simulink model "CombinedExperiment"  (R2020a)
settings: Solver=FixedStepAuto  StartTime=0.0  StopTime=tsim  FixedStep=baseRate  RelTol=1e-3  EnableMultiTasking=on
values from neighbouring files (symbols this model uses):
  baseRate = 0.1    [Run_Initializer.m]
  drop_states_BLACK = [1.36947387695313,1.22175756835938,-0.0161599479615688]    [Run_Initializer.m]
  drop_states_BLUE = [ xLength/2+0.9; yLength/2+0.5; 0]    [Run_Initializer.m]
  drop_states_RED = [ xLength/2+1.1; yLength/2; pi]    [Run_Initializer.m]
  F_thrusters_BLACK = 0.25.*ones(8,1)    [Run_Initializer.m]
  F_thrusters_BLUE = 0.25.*ones(8,1)    [Run_Initializer.m]
  F_thrusters_RED = 0.25.*ones(8,1)    [Run_Initializer.m]
  home_states_BLACK = [ xLength/2; yLength/2; 0]    [Run_Initializer.m]
  home_states_BLUE = [ xLength/2-0.9; yLength/2+0.5; 0]    [Run_Initializer.m]
  home_states_RED = [ xLength/2+1.1; yLength/2; pi]    [Run_Initializer.m]
  init_states_BLACK = [ xLength/2; yLength/2; 0]    [Run_Initializer.m]
  init_states_BLUE = [ xLength/2+0.9; yLength/2+0.5; 0]    [Run_Initializer.m]
  init_states_RED = [ xLength/2+1.1; yLength/2; pi]    [Run_Initializer.m]
  Kd_tb = 0.4    [Run_Initializer.m]
  Kd_tblue = 0.4    [Run_Initializer.m]
  Kd_tr = 0.4    [Run_Initializer.m]
  Kd_xb = 5    [Run_Initializer.m]
  Kd_xblue = 5    [Run_Initializer.m]
  Kd_xr = 5    [Run_Initializer.m]
  Kd_yb = 5    [Run_Initializer.m]
  Kd_yblue = 5    [Run_Initializer.m]
  Kd_yr = 5    [Run_Initializer.m]
  Kp_tb = 0.1    [Run_Initializer.m]
  Kp_tblue = 0.1    [Run_Initializer.m]
  Kp_tr = 0.1    [Run_Initializer.m]
  Kp_xb = 2    [Run_Initializer.m]
  Kp_xblue = 2    [Run_Initializer.m]
  Kp_xr = 2    [Run_Initializer.m]
  Kp_yb = 2    [Run_Initializer.m]
  Kp_yblue = 2    [Run_Initializer.m]
  Kp_yr = 2    [Run_Initializer.m]
  noise_variance_BLACK = 0    [Run_Initializer.m]
  noise_variance_BLUE = 0    [Run_Initializer.m]
  noise_variance_RED = 0    [Run_Initializer.m]
  Phase0_End = Phase0_Duration    (= 10)    [Run_Initializer.m]
  Phase1_End = Phase0_Duration + Phase1_Duration    (= 15)    [Run_Initializer.m]
  Phase2_End = Phase0_Duration + Phase1_Duration +                                   Phase2_Duration    (= 40)    [Run_Initializer.m]
  Phase3_End = Phase0_Duration + Phase1_Duration +                                   Phase2_Duration + Phase3_Duration    (= 117)    [Run_Initializer.m]
  Phase3_SubPhase1_End = Phase2_End + Phase3_SubPhase1_Duration    (= 41)    [Run_Initializer.m]
  Phase3_SubPhase2_End = Phase2_End + Phase3_SubPhase1_Duration +                                   Phase3_SubPhase2_Duration    (= 42)    [Run_Initializer.m]
  Phase3_SubPhase3_End = Phase2_End + Phase3_SubPhase1_Duration +                                   Phase3_SubPhase2_Duration +                                  Phase3_SubPhase3_Duration    (= 72)    [Run_Initializer.m]
  Phase3_SubPhase4_End = Phase2_End + Phase3_SubPhase1_Duration +                                   Phase3_SubPhase2_Duration +                                  Phase3_SubPhase3_Duration +                                  Phase3_SubPhase4_Duration    [Run_Initializer.m]
  Phase4_End = Phase0_Duration + Phase1_Duration +                                   Phase2_Duration + Phase3_Duration +                                   Phase4_Duration    (= 137)    [Run_Initializer.m]
  Phase5_End = Phase0_Duration + Phase1_Duration +                                   Phase2_Duration + Phase3_Duration +                                   Phase4_Duration + Phase5_Duration    (= 142)    [Run_Initializer.m]
  serverRate = 0.2    [Run_Initializer.m]
  thruster_dist2CG_BLACK = [83.42;-52.58;55.94;-60.05;54.08;-53.92;77.06;-55.94]    [Run_Initializer.m]
  thruster_dist2CG_BLUE = [83.42;-52.58;55.94;-60.05;54.08;-53.92;77.06;-55.94]    [Run_Initializer.m]
  thruster_dist2CG_RED = [49.92;-78.08;70.46;-63.54;81.08;-50.42;57.44;-75.96]    [Run_Initializer.m]
  xLength = 3.51155    [Run_Initializer.m]
  yLength = 2.41935    [Run_Initializer.m]
undefined symbols (not defined in the file or in its folder): DiscIntNeverNeededParam, platformSelection, simMode, WhoAmI
libraries: dspstat3 x18, raspberrypiBasiclib x10, dspsigops x9, embdlinuxlib x8, simulink x8, MainLibrary x5, mspfiltlib x3, dsparch4 x3, dspswit3 x2, sensehatlib x1
(part 8 of 9)

== system CombinedExperiment/Gyroscope & Acceleration Algorithms/Change BLUE Behavior/Fix Initial Bias (Accel)/Correct AccelZ/Subsystem ==
  Universal_Time : DataStoreRead  DataStoreName=Univ_Time
  Time : Outport  VectorParamsAs1DForOutWhenUnconnected=off
  wires:
  Universal_Time/1 -> Time/1

== system CombinedExperiment/Gyroscope & Acceleration Algorithms/Change RED Behavior/Fix Initial Bias/Correct GyroX/Calculate Running Mean ==
  In1 : Inport
  Action Port : ActionPort  ActionPortLabel=if(u1 < 5)
  Delay : Delay  DelayLength=1
  Delay1 : Delay
  Delay2 : Delay  DelayLength=4
  Delay3 : Delay  DelayLength=5
  Delay4 : Delay  DelayLength=3
  Mean : dspstat3/Mean  run=off  InputProcessing=Columns as channels (frame based)  reset_popup=None  directionMode=Each column  dimension=1  roiEnable=off  roiType=Rectangles  roiPortion=Entire ROI  roiOutput=Individual statistics for each ROI  roiFlag=off  roundingMode=Floor  overflowMode=off  outputDataTypeStr=Inherit: Same as accumulator  outputMin=[]  outputMax=[]  outputLastDataTypeStr=Inherit: Same as accumulator
  Mux : Mux  Inputs=6
  Out1 : Outport
  wires:
  Delay3/1 -> Mux/6
  Delay2/1 -> Mux/5
  Delay1/1 -> Mux/3
  Delay4/1 -> Mux/4
  Delay/1 -> Mux/2
  In1/1 -> Delay3/1, Delay2/1, Delay4/1, Delay1/1, Delay/1, Mux/1
  Mux/1 -> Mean/1
  Mean/1 -> Out1/1

== system CombinedExperiment/Gyroscope & Acceleration Algorithms/Change RED Behavior/Fix Initial Bias/Correct GyroX/Pass Current Gyro ==
  In1 : Inport
  Action Port : ActionPort  ActionPortLabel=else
  Out1 : Outport
  wires:
  In1/1 -> Out1/1

== system CombinedExperiment/Gyroscope & Acceleration Algorithms/Change RED Behavior/Fix Initial Bias/Correct GyroX/Subsystem ==
  Universal_Time : DataStoreRead  DataStoreName=Univ_Time
  Time : Outport  VectorParamsAs1DForOutWhenUnconnected=off
  wires:
  Universal_Time/1 -> Time/1

== system CombinedExperiment/Gyroscope & Acceleration Algorithms/Change RED Behavior/Fix Initial Bias/Correct GyroY/Calculate Running Mean ==
  In1 : Inport
  Action Port : ActionPort  ActionPortLabel=if(u1 < 5)
  Delay : Delay  DelayLength=1
  Delay1 : Delay
  Delay2 : Delay  DelayLength=4
  Delay3 : Delay  DelayLength=5
  Delay4 : Delay  DelayLength=3
  Mean : dspstat3/Mean  run=off  InputProcessing=Columns as channels (frame based)  reset_popup=None  directionMode=Each column  dimension=1  roiEnable=off  roiType=Rectangles  roiPortion=Entire ROI  roiOutput=Individual statistics for each ROI  roiFlag=off  roundingMode=Floor  overflowMode=off  outputDataTypeStr=Inherit: Same as accumulator  outputMin=[]  outputMax=[]  outputLastDataTypeStr=Inherit: Same as accumulator
  Mux : Mux  Inputs=6
  Out1 : Outport
  wires:
  Delay3/1 -> Mux/6
  Delay2/1 -> Mux/5
  Delay1/1 -> Mux/3
  Delay4/1 -> Mux/4
  Delay/1 -> Mux/2
  In1/1 -> Delay3/1, Delay2/1, Delay4/1, Delay1/1, Delay/1, Mux/1
  Mux/1 -> Mean/1
  Mean/1 -> Out1/1

== system CombinedExperiment/Gyroscope & Acceleration Algorithms/Change RED Behavior/Fix Initial Bias/Correct GyroY/Pass Current Gyro ==
  In1 : Inport
  Action Port : ActionPort  ActionPortLabel=else
  Out1 : Outport
  wires:
  In1/1 -> Out1/1

== system CombinedExperiment/Gyroscope & Acceleration Algorithms/Change RED Behavior/Fix Initial Bias/Correct GyroY/Subsystem ==
  Universal_Time : DataStoreRead  DataStoreName=Univ_Time
  Time : Outport  VectorParamsAs1DForOutWhenUnconnected=off
  wires:
  Universal_Time/1 -> Time/1

== system CombinedExperiment/Gyroscope & Acceleration Algorithms/Change RED Behavior/Fix Initial Bias/Correct GyroZ/Calculate Running Mean ==
  In1 : Inport
  Action Port : ActionPort  ActionPortLabel=if(u1 < 5)
  Delay : Delay  DelayLength=1
  Delay1 : Delay
  Delay2 : Delay  DelayLength=4
  Delay3 : Delay  DelayLength=5
  Delay4 : Delay  DelayLength=3
  Mean : dspstat3/Mean  run=off  InputProcessing=Columns as channels (frame based)  reset_popup=None  directionMode=Each column  dimension=1  roiEnable=off  roiType=Rectangles  roiPortion=Entire ROI  roiOutput=Individual statistics for each ROI  roiFlag=off  roundingMode=Floor  overflowMode=off  outputDataTypeStr=Inherit: Same as accumulator  outputMin=[]  outputMax=[]  outputLastDataTypeStr=Inherit: Same as accumulator
  Mux : Mux  Inputs=6
  Out1 : Outport
  wires:
  Delay3/1 -> Mux/6
  Delay2/1 -> Mux/5
  Delay1/1 -> Mux/3
  Delay4/1 -> Mux/4
  Delay/1 -> Mux/2
  In1/1 -> Delay3/1, Delay2/1, Delay4/1, Delay1/1, Delay/1, Mux/1
  Mux/1 -> Mean/1
  Mean/1 -> Out1/1

== system CombinedExperiment/Gyroscope & Acceleration Algorithms/Change RED Behavior/Fix Initial Bias/Correct GyroZ/Pass Current Gyro ==
  In1 : Inport
  Action Port : ActionPort  ActionPortLabel=else
  Out1 : Outport
  wires:
  In1/1 -> Out1/1

== system CombinedExperiment/Gyroscope & Acceleration Algorithms/Change RED Behavior/Fix Initial Bias/Correct GyroZ/Subsystem ==
  Universal_Time : DataStoreRead  DataStoreName=Univ_Time
  Time : Outport  VectorParamsAs1DForOutWhenUnconnected=off
  wires:
  Universal_Time/1 -> Time/1

== system CombinedExperiment/Gyroscope & Acceleration Algorithms/Change RED Behavior/Fix Initial Bias (Accel)/Correct AccelX/Calculate Running Mean ==
  In1 : Inport
  Action Port : ActionPort  ActionPortLabel=if(u1 < 5)
  Delay : Delay  DelayLength=1
  Delay1 : Delay
  Delay2 : Delay  DelayLength=4
  Delay3 : Delay  DelayLength=5
  Delay4 : Delay  DelayLength=3
  Mean : dspstat3/Mean  run=off  InputProcessing=Columns as channels (frame based)  reset_popup=None  directionMode=Each column  dimension=1  roiEnable=off  roiType=Rectangles  roiPortion=Entire ROI  roiOutput=Individual statistics for each ROI  roiFlag=off  roundingMode=Floor  overflowMode=off  outputDataTypeStr=Inherit: Same as accumulator  outputMin=[]  outputMax=[]  outputLastDataTypeStr=Inherit: Same as accumulator
  Mux : Mux  Inputs=6
  Out1 : Outport
  wires:
  Delay3/1 -> Mux/6
  Delay2/1 -> Mux/5
  Delay1/1 -> Mux/3
  Delay4/1 -> Mux/4
  Delay/1 -> Mux/2
  In1/1 -> Delay3/1, Delay2/1, Delay4/1, Delay1/1, Delay/1, Mux/1
  Mux/1 -> Mean/1
  Mean/1 -> Out1/1

== system CombinedExperiment/Gyroscope & Acceleration Algorithms/Change RED Behavior/Fix Initial Bias (Accel)/Correct AccelX/Pass Current Accel ==
  In1 : Inport
  Action Port : ActionPort  ActionPortLabel=else
  Out1 : Outport
  wires:
  In1/1 -> Out1/1

== system CombinedExperiment/Gyroscope & Acceleration Algorithms/Change RED Behavior/Fix Initial Bias (Accel)/Correct AccelX/Subsystem ==
  Universal_Time : DataStoreRead  DataStoreName=Univ_Time
  Time : Outport  VectorParamsAs1DForOutWhenUnconnected=off
  wires:
  Universal_Time/1 -> Time/1

== system CombinedExperiment/Gyroscope & Acceleration Algorithms/Change RED Behavior/Fix Initial Bias (Accel)/Correct AccelY/Calculate Running Mean ==
  In1 : Inport
  Action Port : ActionPort  ActionPortLabel=if(u1 < 5)
  Delay : Delay  DelayLength=1
  Delay1 : Delay
  Delay2 : Delay  DelayLength=4
  Delay3 : Delay  DelayLength=5
  Delay4 : Delay  DelayLength=3
  Mean : dspstat3/Mean  run=off  InputProcessing=Columns as channels (frame based)  reset_popup=None  directionMode=Each column  dimension=1  roiEnable=off  roiType=Rectangles  roiPortion=Entire ROI  roiOutput=Individual statistics for each ROI  roiFlag=off  roundingMode=Floor  overflowMode=off  outputDataTypeStr=Inherit: Same as accumulator  outputMin=[]  outputMax=[]  outputLastDataTypeStr=Inherit: Same as accumulator
  Mux : Mux  Inputs=6
  Out1 : Outport
  wires:
  Delay3/1 -> Mux/6
  Delay2/1 -> Mux/5
  Delay1/1 -> Mux/3
  Delay4/1 -> Mux/4
  Delay/1 -> Mux/2
  In1/1 -> Delay3/1, Delay2/1, Delay4/1, Delay1/1, Delay/1, Mux/1
  Mux/1 -> Mean/1
  Mean/1 -> Out1/1

== system CombinedExperiment/Gyroscope & Acceleration Algorithms/Change RED Behavior/Fix Initial Bias (Accel)/Correct AccelY/Pass Current Accel ==
  In1 : Inport
  Action Port : ActionPort  ActionPortLabel=else
  Out1 : Outport
  wires:
  In1/1 -> Out1/1

== system CombinedExperiment/Gyroscope & Acceleration Algorithms/Change RED Behavior/Fix Initial Bias (Accel)/Correct AccelY/Subsystem ==
  Universal_Time : DataStoreRead  DataStoreName=Univ_Time
  Time : Outport  VectorParamsAs1DForOutWhenUnconnected=off
  wires:
  Universal_Time/1 -> Time/1

== system CombinedExperiment/Gyroscope & Acceleration Algorithms/Change RED Behavior/Fix Initial Bias (Accel)/Correct AccelZ/Calculate Running Mean ==
  In1 : Inport
  Action Port : ActionPort  ActionPortLabel=if(u1 < 5)
  Constant : Constant  Value=9.81
  Delay : Delay  DelayLength=1
  Delay1 : Delay
  Delay2 : Delay  DelayLength=4
  Delay3 : Delay  DelayLength=5
  Delay4 : Delay  DelayLength=3
  Mean : dspstat3/Mean  run=off  InputProcessing=Columns as channels (frame based)  reset_popup=None  directionMode=Each column  dimension=1  roiEnable=off  roiType=Rectangles  roiPortion=Entire ROI  roiOutput=Individual statistics for each ROI  roiFlag=off  roundingMode=Floor  overflowMode=off  outputDataTypeStr=Inherit: Same as accumulator  outputMin=[]  outputMax=[]  outputLastDataTypeStr=Inherit: Same as accumulator
  Mux : Mux  Inputs=6
  Subtract : Sum  Inputs=+-
  Out1 : Outport
  wires:
  Delay3/1 -> Mux/6
  Delay2/1 -> Mux/5
  Delay1/1 -> Mux/3
  Delay4/1 -> Mux/4
  Delay/1 -> Mux/2
  In1/1 -> Delay3/1, Delay2/1, Delay4/1, Delay1/1, Delay/1, Mux/1
  Mux/1 -> Mean/1
  Subtract/1 -> Out1/1
  Mean/1 -> Subtract/1
  Constant/1 -> Subtract/2

== system CombinedExperiment/Gyroscope & Acceleration Algorithms/Change RED Behavior/Fix Initial Bias (Accel)/Correct AccelZ/Pass Current Accel ==
  In1 : Inport
  Action Port : ActionPort  ActionPortLabel=else
  Out1 : Outport
  wires:
  In1/1 -> Out1/1

== system CombinedExperiment/Gyroscope & Acceleration Algorithms/Change RED Behavior/Fix Initial Bias (Accel)/Correct AccelZ/Subsystem ==
  Universal_Time : DataStoreRead  DataStoreName=Univ_Time
  Time : Outport  VectorParamsAs1DForOutWhenUnconnected=off
  wires:
  Universal_Time/1 -> Time/1

== system CombinedExperiment/Phase #2: Move to Initial Position/Change BLACK Behavior/Custom Discrete PD (Attitude)/x_dot -> x1/Hold this value ==
  In1 : Inport
  Action Port : ActionPort  ActionPortLabel=if(u1 ~= 0)
  Out1 : Outport  VectorParamsAs1DForOutWhenUnconnected=off
  wires:
  In1/1 -> Out1/1

== system CombinedExperiment/Phase #2: Move to Initial Position/Change BLACK Behavior/Custom Discrete PD (X-Position)/x_dot -> x1/Hold this value ==
  In1 : Inport
  Action Port : ActionPort  ActionPortLabel=if(u1 ~= 0)
  Out1 : Outport  VectorParamsAs1DForOutWhenUnconnected=off
  wires:
  In1/1 -> Out1/1

== system CombinedExperiment/Phase #2: Move to Initial Position/Change BLACK Behavior/Custom Discrete PD (Y-Position)/x_dot -> x1/Hold this value ==
  In1 : Inport
  Action Port : ActionPort  ActionPortLabel=if(u1 ~= 0)
  Out1 : Outport  VectorParamsAs1DForOutWhenUnconnected=off
  wires:
  In1/1 -> Out1/1

== system CombinedExperiment/Phase #2: Move to Initial Position/Change BLUE Behavior/Custom Discrete PD (Attitude)/x_dot -> x1/Hold this value ==
  In1 : Inport
  Action Port : ActionPort  ActionPortLabel=if(u1 ~= 0)
  Out1 : Outport  VectorParamsAs1DForOutWhenUnconnected=off
  wires:
  In1/1 -> Out1/1

== system CombinedExperiment/Phase #2: Move to Initial Position/Change BLUE Behavior/Custom Discrete PD (X-Position)/x_dot -> x1/Hold this value ==
  In1 : Inport
  Action Port : ActionPort  ActionPortLabel=if(u1 ~= 0)
  Out1 : Outport  VectorParamsAs1DForOutWhenUnconnected=off
  wires:
  In1/1 -> Out1/1

== system CombinedExperiment/Phase #2: Move to Initial Position/Change BLUE Behavior/Custom Discrete PD (Y-Position)/x_dot -> x1/Hold this value ==
  In1 : Inport
  Action Port : ActionPort  ActionPortLabel=if(u1 ~= 0)
  Out1 : Outport  VectorParamsAs1DForOutWhenUnconnected=off
  wires:
  In1/1 -> Out1/1

== system CombinedExperiment/Phase #2: Move to Initial Position/Change RED Behavior/Custom Discrete PD (Attitude)/x_dot -> x1/Hold this value ==
  In1 : Inport
  Action Port : ActionPort  ActionPortLabel=if(u1 ~= 0)
  Out1 : Outport  VectorParamsAs1DForOutWhenUnconnected=off
  wires:
  In1/1 -> Out1/1

== system CombinedExperiment/Phase #2: Move to Initial Position/Change RED Behavior/Custom Discrete PD (X-Position)/x_dot -> x1/Hold this value ==
  In1 : Inport
  Action Port : ActionPort  ActionPortLabel=if(u1 ~= 0)
  Out1 : Outport  VectorParamsAs1DForOutWhenUnconnected=off
  wires:
  In1/1 -> Out1/1

== system CombinedExperiment/Phase #2: Move to Initial Position/Change RED Behavior/Custom Discrete PD (Y-Position)/x_dot -> x1/Hold this value ==
  In1 : Inport
  Action Port : ActionPort  ActionPortLabel=if(u1 ~= 0)
  Out1 : Outport  VectorParamsAs1DForOutWhenUnconnected=off
  wires:
  In1/1 -> Out1/1

== system CombinedExperiment/Phase #3: Experiment/Change BLACK Behavior/Sub-Phase #1/Custom Discrete PD (Attitude)/x_dot -> x1 ==
  note: dy/dt ~= (y2-y1)/deltaT
  y(t) : Inport
  Delay1 : Delay  DelayLength=1  InitialConditionSource=Input port
      settings: InputPortMap=u0,p4
  Hold this value : Subsystem  TreatAsAtomicUnit=on
  Sum6 : Sum  Inputs=-+|
  divide by delta T : Gain  Gain=1/serverRate
  "if we went through a \"step\"" : If  IfExpression=u1 ~= 0  ShowElse=off
  dy(t)/dt : Outport  VectorParamsAs1DForOutWhenUnconnected=off
  wires:
  divide by delta T/1 -> dy(t)/dt/1
  Delay1/1 -> Sum6/1
  "if we went through a \"step\""/1 -> Hold this value/Action
  Hold this value/1(Out1) -> divide by delta T/1
  Sum6/1 -> "if we went through a \"step\""/1, Hold this value/1(In1)
  y(t)/1 -> Sum6/2, Delay1/2, Delay1/1

== system CombinedExperiment/Phase #3: Experiment/Change BLACK Behavior/Sub-Phase #1/Custom Discrete PD (X-Position)/x_dot -> x1 ==
  note: dy/dt ~= (y2-y1)/deltaT
  y(t) : Inport
  Delay1 : Delay  DelayLength=1  InitialConditionSource=Input port
      settings: InputPortMap=u0,p4
  Hold this value : Subsystem  TreatAsAtomicUnit=on
  Sum6 : Sum  Inputs=-+|
  divide by delta T : Gain  Gain=1/serverRate
  "if we went through a \"step\"" : If  IfExpression=u1 ~= 0  ShowElse=off
  dy(t)/dt : Outport  VectorParamsAs1DForOutWhenUnconnected=off
  wires:
  divide by delta T/1 -> dy(t)/dt/1
  Delay1/1 -> Sum6/1
  "if we went through a \"step\""/1 -> Hold this value/Action
  Hold this value/1(Out1) -> divide by delta T/1
  Sum6/1 -> "if we went through a \"step\""/1, Hold this value/1(In1)
  y(t)/1 -> Sum6/2, Delay1/2, Delay1/1

== system CombinedExperiment/Phase #3: Experiment/Change BLACK Behavior/Sub-Phase #1/Custom Discrete PD (Y-Position)/x_dot -> x1 ==
  note: dy/dt ~= (y2-y1)/deltaT
  y(t) : Inport
  Delay1 : Delay  DelayLength=1  InitialConditionSource=Input port
      settings: InputPortMap=u0,p4
  Hold this value : Subsystem  TreatAsAtomicUnit=on
  Sum6 : Sum  Inputs=-+|
  divide by delta T : Gain  Gain=1/serverRate
  "if we went through a \"step\"" : If  IfExpression=u1 ~= 0  ShowElse=off
  dy(t)/dt : Outport  VectorParamsAs1DForOutWhenUnconnected=off
  wires:
  divide by delta T/1 -> dy(t)/dt/1
  Delay1/1 -> Sum6/1
  "if we went through a \"step\""/1 -> Hold this value/Action
  Hold this value/1(Out1) -> divide by delta T/1
  Sum6/1 -> "if we went through a \"step\""/1, Hold this value/1(In1)
  y(t)/1 -> Sum6/2, Delay1/2, Delay1/1

== system CombinedExperiment/Phase #3: Experiment/Change BLACK Behavior/Sub-Phase #4/BLACK_RzD/Subsystem ==
  Constant1 : Constant  Value=Phase3_SubPhase3_End  SampleTime=-1
  Subtract : Sum  Inputs=+-
  Universal_Time : DataStoreRead  DataStoreName=Univ_Time
  Time : Outport  VectorParamsAs1DForOutWhenUnconnected=off
  wires:
  Universal_Time/1 -> Subtract/1
  Subtract/1 -> Time/1
  Constant1/1 -> Subtract/2

== system CombinedExperiment/Phase #3: Experiment/Change BLACK Behavior/Sub-Phase #4/BLACK_RzD/Wrap1 ==
  unwrapped : Inport
  MATLAB Function : MATLAB Function  TreatAsAtomicUnit=on
  wrapped : Outport  VectorParamsAs1DForOutWhenUnconnected=off
  wires:
  MATLAB Function/1(wrappedAngle) -> wrapped/1
  unwrapped/1 -> MATLAB Function/1(u)

== system CombinedExperiment/Phase #3: Experiment/Change BLACK Behavior/Sub-Phase #4/BLACK_RzD1/Subsystem ==
  Constant1 : Constant  Value=Phase3_SubPhase3_End  SampleTime=-1
  Subtract : Sum  Inputs=+-
  Universal_Time : DataStoreRead  DataStoreName=Univ_Time
  Time : Outport  VectorParamsAs1DForOutWhenUnconnected=off
  wires:
  Universal_Time/1 -> Subtract/1
  Subtract/1 -> Time/1
  Constant1/1 -> Subtract/2

== system CombinedExperiment/Phase #3: Experiment/Change BLACK Behavior/Sub-Phase #4/BLACK_RzD1/Wrap1 ==
  unwrapped : Inport
  MATLAB Function : MATLAB Function  TreatAsAtomicUnit=on
  wrapped : Outport  VectorParamsAs1DForOutWhenUnconnected=off
  wires:
  MATLAB Function/1(wrappedAngle) -> wrapped/1
  unwrapped/1 -> MATLAB Function/1(u)

== system CombinedExperiment/Phase #3: Experiment/Change BLACK Behavior/Sub-Phase #4/Custom Discrete PD (Attitude)/x_dot -> x1 ==
  note: dy/dt ~= (y2-y1)/deltaT
  y(t) : Inport
  Delay1 : Delay  DelayLength=1  InitialConditionSource=Input port
      settings: InputPortMap=u0,p4
  Hold this value : Subsystem  TreatAsAtomicUnit=on
  Sum6 : Sum  Inputs=-+|
  divide by delta T : Gain  Gain=1/serverRate
  "if we went through a \"step\"" : If  IfExpression=u1 ~= 0  ShowElse=off
  dy(t)/dt : Outport  VectorParamsAs1DForOutWhenUnconnected=off
  wires:
  divide by delta T/1 -> dy(t)/dt/1
  Delay1/1 -> Sum6/1
  "if we went through a \"step\""/1 -> Hold this value/Action
  Hold this value/1(Out1) -> divide by delta T/1
  Sum6/1 -> "if we went through a \"step\""/1, Hold this value/1(In1)
  y(t)/1 -> Sum6/2, Delay1/2, Delay1/1

== system CombinedExperiment/Phase #3: Experiment/Change BLACK Behavior/Sub-Phase #4/Custom Discrete PD (X-Position)/x_dot -> x1 ==
  note: dy/dt ~= (y2-y1)/deltaT
  y(t) : Inport
  Delay1 : Delay  DelayLength=1  InitialConditionSource=Input port
      settings: InputPortMap=u0,p4
  Hold this value : Subsystem  TreatAsAtomicUnit=on
  Sum6 : Sum  Inputs=-+|
  divide by delta T : Gain  Gain=1/serverRate
  "if we went through a \"step\"" : If  IfExpression=u1 ~= 0  ShowElse=off
  dy(t)/dt : Outport  VectorParamsAs1DForOutWhenUnconnected=off
  wires:
  divide by delta T/1 -> dy(t)/dt/1
  Delay1/1 -> Sum6/1
  "if we went through a \"step\""/1 -> Hold this value/Action
  Hold this value/1(Out1) -> divide by delta T/1
  Sum6/1 -> "if we went through a \"step\""/1, Hold this value/1(In1)
  y(t)/1 -> Sum6/2, Delay1/2, Delay1/1

== system CombinedExperiment/Phase #3: Experiment/Change BLACK Behavior/Sub-Phase #4/Custom Discrete PD (Y-Position)/x_dot -> x1 ==
  note: dy/dt ~= (y2-y1)/deltaT
  y(t) : Inport
  Delay1 : Delay  DelayLength=1  InitialConditionSource=Input port
      settings: InputPortMap=u0,p4
  Hold this value : Subsystem  TreatAsAtomicUnit=on
  Sum6 : Sum  Inputs=-+|
  divide by delta T : Gain  Gain=1/serverRate
  "if we went through a \"step\"" : If  IfExpression=u1 ~= 0  ShowElse=off
  dy(t)/dt : Outport  VectorParamsAs1DForOutWhenUnconnected=off
  wires:
  divide by delta T/1 -> dy(t)/dt/1
  Delay1/1 -> Sum6/1
  "if we went through a \"step\""/1 -> Hold this value/Action
  Hold this value/1(Out1) -> divide by delta T/1
  Sum6/1 -> "if we went through a \"step\""/1, Hold this value/1(In1)
  y(t)/1 -> Sum6/2, Delay1/2, Delay1/1

== system CombinedExperiment/Phase #3: Experiment/Change BLUE Behavior/Sub-Phase #1/Custom Discrete PD (Attitude)/x_dot -> x1 ==
  note: dy/dt ~= (y2-y1)/deltaT
  y(t) : Inport
  Delay1 : Delay  DelayLength=1  InitialConditionSource=Input port
      settings: InputPortMap=u0,p4
  Hold this value : Subsystem  TreatAsAtomicUnit=on
  Sum6 : Sum  Inputs=-+|
  divide by delta T : Gain  Gain=1/serverRate
  "if we went through a \"step\"" : If  IfExpression=u1 ~= 0  ShowElse=off
  dy(t)/dt : Outport  VectorParamsAs1DForOutWhenUnconnected=off
  wires:
  divide by delta T/1 -> dy(t)/dt/1
  Delay1/1 -> Sum6/1
  "if we went through a \"step\""/1 -> Hold this value/Action
  Hold this value/1(Out1) -> divide by delta T/1
  Sum6/1 -> "if we went through a \"step\""/1, Hold this value/1(In1)
  y(t)/1 -> Sum6/2, Delay1/2, Delay1/1

== system CombinedExperiment/Phase #3: Experiment/Change BLUE Behavior/Sub-Phase #1/Custom Discrete PD (X-Position)/x_dot -> x1 ==
  note: dy/dt ~= (y2-y1)/deltaT
  y(t) : Inport
  Delay1 : Delay  DelayLength=1  InitialConditionSource=Input port
      settings: InputPortMap=u0,p4
  Hold this value : Subsystem  TreatAsAtomicUnit=on
  Sum6 : Sum  Inputs=-+|
  divide by delta T : Gain  Gain=1/serverRate
  "if we went through a \"step\"" : If  IfExpression=u1 ~= 0  ShowElse=off
  dy(t)/dt : Outport  VectorParamsAs1DForOutWhenUnconnected=off
  wires:
  divide by delta T/1 -> dy(t)/dt/1
  Delay1/1 -> Sum6/1
  "if we went through a \"step\""/1 -> Hold this value/Action
  Hold this value/1(Out1) -> divide by delta T/1
  Sum6/1 -> "if we went through a \"step\""/1, Hold this value/1(In1)
  y(t)/1 -> Sum6/2, Delay1/2, Delay1/1

== system CombinedExperiment/Phase #3: Experiment/Change BLUE Behavior/Sub-Phase #1/Custom Discrete PD (Y-Position)/x_dot -> x1 ==
  note: dy/dt ~= (y2-y1)/deltaT
  y(t) : Inport
  Delay1 : Delay  DelayLength=1  InitialConditionSource=Input port
      settings: InputPortMap=u0,p4
  Hold this value : Subsystem  TreatAsAtomicUnit=on
  Sum6 : Sum  Inputs=-+|
  divide by delta T : Gain  Gain=1/serverRate
  "if we went through a \"step\"" : If  IfExpression=u1 ~= 0  ShowElse=off
  dy(t)/dt : Outport  VectorParamsAs1DForOutWhenUnconnected=off
  wires:
  divide by delta T/1 -> dy(t)/dt/1
  Delay1/1 -> Sum6/1
  "if we went through a \"step\""/1 -> Hold this value/Action
  Hold this value/1(Out1) -> divide by delta T/1
  Sum6/1 -> "if we went through a \"step\""/1, Hold this value/1(In1)
  y(t)/1 -> Sum6/2, Delay1/2, Delay1/1

== system CombinedExperiment/Phase #3: Experiment/Change BLUE Behavior/Sub-Phase #4/Custom Discrete PD (Attitude)/x_dot -> x1 ==
  note: dy/dt ~= (y2-y1)/deltaT
  y(t) : Inport
  Delay1 : Delay  DelayLength=1  InitialConditionSource=Input port
      settings: InputPortMap=u0,p4
  Hold this value : Subsystem  TreatAsAtomicUnit=on
  Sum6 : Sum  Inputs=-+|
  divide by delta T : Gain  Gain=1/serverRate
  "if we went through a \"step\"" : If  IfExpression=u1 ~= 0  ShowElse=off
  dy(t)/dt : Outport  VectorParamsAs1DForOutWhenUnconnected=off
  wires:
  divide by delta T/1 -> dy(t)/dt/1
  Delay1/1 -> Sum6/1
  "if we went through a \"step\""/1 -> Hold this value/Action
  Hold this value/1(Out1) -> divide by delta T/1
  Sum6/1 -> "if we went through a \"step\""/1, Hold this value/1(In1)
  y(t)/1 -> Sum6/2, Delay1/2, Delay1/1

== system CombinedExperiment/Phase #3: Experiment/Change BLUE Behavior/Sub-Phase #4/Custom Discrete PD (X-Position)/x_dot -> x1 ==
  note: dy/dt ~= (y2-y1)/deltaT
  y(t) : Inport
  Delay1 : Delay  DelayLength=1  InitialConditionSource=Input port
      settings: InputPortMap=u0,p4
  Hold this value : Subsystem  TreatAsAtomicUnit=on
  Sum6 : Sum  Inputs=-+|
  divide by delta T : Gain  Gain=1/serverRate
  "if we went through a \"step\"" : If  IfExpression=u1 ~= 0  ShowElse=off
  dy(t)/dt : Outport  VectorParamsAs1DForOutWhenUnconnected=off
  wires:
  divide by delta T/1 -> dy(t)/dt/1
  Delay1/1 -> Sum6/1
  "if we went through a \"step\""/1 -> Hold this value/Action
  Hold this value/1(Out1) -> divide by delta T/1
  Sum6/1 -> "if we went through a \"step\""/1, Hold this value/1(In1)
  y(t)/1 -> Sum6/2, Delay1/2, Delay1/1

== system CombinedExperiment/Phase #3: Experiment/Change BLUE Behavior/Sub-Phase #4/Custom Discrete PD (Y-Position)/x_dot -> x1 ==
  note: dy/dt ~= (y2-y1)/deltaT
  y(t) : Inport
  Delay1 : Delay  DelayLength=1  InitialConditionSource=Input port
      settings: InputPortMap=u0,p4
  Hold this value : Subsystem  TreatAsAtomicUnit=on
  Sum6 : Sum  Inputs=-+|
  divide by delta T : Gain  Gain=1/serverRate
  "if we went through a \"step\"" : If  IfExpression=u1 ~= 0  ShowElse=off
  dy(t)/dt : Outport  VectorParamsAs1DForOutWhenUnconnected=off
  wires:
  divide by delta T/1 -> dy(t)/dt/1
  Delay1/1 -> Sum6/1
  "if we went through a \"step\""/1 -> Hold this value/Action
  Hold this value/1(Out1) -> divide by delta T/1
  Sum6/1 -> "if we went through a \"step\""/1, Hold this value/1(In1)
  y(t)/1 -> Sum6/2, Delay1/2, Delay1/1

== system CombinedExperiment/Phase #3: Experiment/Change RED Behavior/Sub-Phase #4/Custom Discrete PD (Attitude)2/x_dot -> x1 ==
  note: dy/dt ~= (y2-y1)/deltaT
  y(t) : Inport
  Delay1 : Delay  DelayLength=1  InitialConditionSource=Input port
      settings: InputPortMap=u0,p4
  Hold this value : Subsystem  TreatAsAtomicUnit=on
  Sum6 : Sum  Inputs=-+|
  divide by delta T : Gain  Gain=1/serverRate
  "if we went through a \"step\"" : If  IfExpression=u1 ~= 0  ShowElse=off
  dy(t)/dt : Outport  VectorParamsAs1DForOutWhenUnconnected=off
  wires:
  divide by delta T/1 -> dy(t)/dt/1
  Delay1/1 -> Sum6/1
  "if we went through a \"step\""/1 -> Hold this value/Action
  Hold this value/1(Out1) -> divide by delta T/1
  Sum6/1 -> "if we went through a \"step\""/1, Hold this value/1(In1)
  y(t)/1 -> Sum6/2, Delay1/2, Delay1/1

== system CombinedExperiment/Phase #3: Experiment/Change RED Behavior/Sub-Phase #4/x_dot -> x1/Hold this value ==
  In1 : Inport
  Action Port : ActionPort  ActionPortLabel=if(u1 ~= 0)
  Out1 : Outport  VectorParamsAs1DForOutWhenUnconnected=off
  wires:
  In1/1 -> Out1/1

== system CombinedExperiment/Phase #3: Experiment/Change RED Behavior/Sub-Phase #4/x_dot -> x2/Hold this value ==
  In1 : Inport
  Action Port : ActionPort  ActionPortLabel=if(u1 ~= 0)
  Out1 : Outport  VectorParamsAs1DForOutWhenUnconnected=off
  wires:
  In1/1 -> Out1/1

== system CombinedExperiment/Phase #4: Return Home/Change BLACK Behavior/Custom Discrete PD (Attitude)/x_dot -> x1/Hold this value ==
  In1 : Inport
  Action Port : ActionPort  ActionPortLabel=if(u1 ~= 0)
  Out1 : Outport  VectorParamsAs1DForOutWhenUnconnected=off
  wires:
  In1/1 -> Out1/1

== system CombinedExperiment/Phase #4: Return Home/Change BLACK Behavior/Custom Discrete PD (X-Position)/x_dot -> x1/Hold this value ==
  In1 : Inport
  Action Port : ActionPort  ActionPortLabel=if(u1 ~= 0)
  Out1 : Outport  VectorParamsAs1DForOutWhenUnconnected=off
  wires:
  In1/1 -> Out1/1

== system CombinedExperiment/Phase #4: Return Home/Change BLACK Behavior/Custom Discrete PD (Y-Position)/x_dot -> x1/Hold this value ==
  In1 : Inport
  Action Port : ActionPort  ActionPortLabel=if(u1 ~= 0)
  Out1 : Outport  VectorParamsAs1DForOutWhenUnconnected=off
  wires:
  In1/1 -> Out1/1

== system CombinedExperiment/Phase #4: Return Home/Change BLUE Behavior/Custom Discrete PD (Attitude)/x_dot -> x1/Hold this value ==
  In1 : Inport
  Action Port : ActionPort  ActionPortLabel=if(u1 ~= 0)
  Out1 : Outport  VectorParamsAs1DForOutWhenUnconnected=off
  wires:
  In1/1 -> Out1/1

== system CombinedExperiment/Phase #4: Return Home/Change BLUE Behavior/Custom Discrete PD (X-Position)/x_dot -> x1/Hold this value ==
  In1 : Inport
  Action Port : ActionPort  ActionPortLabel=if(u1 ~= 0)
  Out1 : Outport  VectorParamsAs1DForOutWhenUnconnected=off
  wires:
  In1/1 -> Out1/1

== system CombinedExperiment/Phase #4: Return Home/Change BLUE Behavior/Custom Discrete PD (Y-Position)/x_dot -> x1/Hold this value ==
  In1 : Inport
  Action Port : ActionPort  ActionPortLabel=if(u1 ~= 0)
  Out1 : Outport  VectorParamsAs1DForOutWhenUnconnected=off
  wires:
  In1/1 -> Out1/1

== system CombinedExperiment/Phase #4: Return Home/Change RED Behavior/Custom Discrete PD (Attitude)/x_dot -> x1/Hold this value ==
  In1 : Inport
  Action Port : ActionPort  ActionPortLabel=if(u1 ~= 0)
  Out1 : Outport  VectorParamsAs1DForOutWhenUnconnected=off
  wires:
  In1/1 -> Out1/1

== system CombinedExperiment/Phase #4: Return Home/Change RED Behavior/Custom Discrete PD (X-Position)/x_dot -> x1/Hold this value ==
  In1 : Inport
  Action Port : ActionPort  ActionPortLabel=if(u1 ~= 0)
  Out1 : Outport  VectorParamsAs1DForOutWhenUnconnected=off
  wires:
  In1/1 -> Out1/1

== system CombinedExperiment/Phase #4: Return Home/Change RED Behavior/Custom Discrete PD (Y-Position)/x_dot -> x1/Hold this value ==
  In1 : Inport
  Action Port : ActionPort  ActionPortLabel=if(u1 ~= 0)
  Out1 : Outport  VectorParamsAs1DForOutWhenUnconnected=off
  wires:
  In1/1 -> Out1/1

== system CombinedExperiment/Phase #5: Hold Home/Change BLACK Behavior/Custom Discrete PD (Attitude)/x_dot -> x1/Hold this value ==
  In1 : Inport
  Action Port : ActionPort  ActionPortLabel=if(u1 ~= 0)
  Out1 : Outport  VectorParamsAs1DForOutWhenUnconnected=off
  wires:
  In1/1 -> Out1/1

== system CombinedExperiment/Phase #5: Hold Home/Change BLACK Behavior/Custom Discrete PD (X-Position)/x_dot -> x1/Hold this value ==
  In1 : Inport
  Action Port : ActionPort  ActionPortLabel=if(u1 ~= 0)
  Out1 : Outport  VectorParamsAs1DForOutWhenUnconnected=off
  wires:
  In1/1 -> Out1/1

== system CombinedExperiment/Phase #5: Hold Home/Change BLACK Behavior/Custom Discrete PD (Y-Position)/x_dot -> x1/Hold this value ==
  In1 : Inport
  Action Port : ActionPort  ActionPortLabel=if(u1 ~= 0)
  Out1 : Outport  VectorParamsAs1DForOutWhenUnconnected=off
  wires:
  In1/1 -> Out1/1

== system CombinedExperiment/Phase #5: Hold Home/Change BLUE Behavior/Custom Discrete PD (Attitude)/x_dot -> x1/Hold this value ==
  In1 : Inport
  Action Port : ActionPort  ActionPortLabel=if(u1 ~= 0)
  Out1 : Outport  VectorParamsAs1DForOutWhenUnconnected=off
  wires:
  In1/1 -> Out1/1

== system CombinedExperiment/Phase #5: Hold Home/Change BLUE Behavior/Custom Discrete PD (X-Position)/x_dot -> x1/Hold this value ==
  In1 : Inport
  Action Port : ActionPort  ActionPortLabel=if(u1 ~= 0)
  Out1 : Outport  VectorParamsAs1DForOutWhenUnconnected=off
  wires:
  In1/1 -> Out1/1

== system CombinedExperiment/Phase #5: Hold Home/Change BLUE Behavior/Custom Discrete PD (Y-Position)/x_dot -> x1/Hold this value ==
  In1 : Inport
  Action Port : ActionPort  ActionPortLabel=if(u1 ~= 0)
  Out1 : Outport  VectorParamsAs1DForOutWhenUnconnected=off
  wires:
  In1/1 -> Out1/1

== system CombinedExperiment/Phase #5: Hold Home/Change RED Behavior/Custom Discrete PD (Attitude)/x_dot -> x1/Hold this value ==
  In1 : Inport
  Action Port : ActionPort  ActionPortLabel=if(u1 ~= 0)
  Out1 : Outport  VectorParamsAs1DForOutWhenUnconnected=off
  wires:
  In1/1 -> Out1/1

== system CombinedExperiment/Phase #5: Hold Home/Change RED Behavior/Custom Discrete PD (X-Position)/x_dot -> x1/Hold this value ==
  In1 : Inport
  Action Port : ActionPort  ActionPortLabel=if(u1 ~= 0)
  Out1 : Outport  VectorParamsAs1DForOutWhenUnconnected=off
  wires:
  In1/1 -> Out1/1

== system CombinedExperiment/Phase #5: Hold Home/Change RED Behavior/Custom Discrete PD (Y-Position)/x_dot -> x1/Hold this value ==
  In1 : Inport
  Action Port : ActionPort  ActionPortLabel=if(u1 ~= 0)
  Out1 : Outport  VectorParamsAs1DForOutWhenUnconnected=off
  wires:
  In1/1 -> Out1/1

== system CombinedExperiment/Grab PhaseSpace Data via UDP/Use Hardware to Obtain States/Using RED+BLACK, or RED+BLACK+ARM/Obtain BLACK States/x_dot -> x1/Hold this value ==
  In1 : Inport
  Action Port : ActionPort  ActionPortLabel=if(u1 ~= 0)
  Out1 : Outport  VectorParamsAs1DForOutWhenUnconnected=off
  wires:
  In1/1 -> Out1/1

== system CombinedExperiment/Grab PhaseSpace Data via UDP/Use Hardware to Obtain States/Using RED+BLACK, or RED+BLACK+ARM/Obtain BLACK States/x_dot -> x10/Hold this value ==
  In1 : Inport
  Action Port : ActionPort  ActionPortLabel=if(u1 ~= 0)
  Out1 : Outport  VectorParamsAs1DForOutWhenUnconnected=off
  wires:
  In1/1 -> Out1/1

== system CombinedExperiment/Grab PhaseSpace Data via UDP/Use Hardware to Obtain States/Using RED+BLACK, or RED+BLACK+ARM/Obtain BLACK States/x_dot -> x11/Hold this value ==
  In1 : Inport
  Action Port : ActionPort  ActionPortLabel=if(u1 ~= 0)
  Out1 : Outport  VectorParamsAs1DForOutWhenUnconnected=off
  wires:
  In1/1 -> Out1/1

== system CombinedExperiment/Grab PhaseSpace Data via UDP/Use Hardware to Obtain States/Using RED+BLACK, or RED+BLACK+ARM/Obtain BLACK States/x_dot -> x12/Hold this value ==
  In1 : Inport
  Action Port : ActionPort  ActionPortLabel=if(u1 ~= 0)
  Out1 : Outport  VectorParamsAs1DForOutWhenUnconnected=off
  wires:
  In1/1 -> Out1/1

== system CombinedExperiment/Grab PhaseSpace Data via UDP/Use Hardware to Obtain States/Using RED+BLACK, or RED+BLACK+ARM/Obtain BLACK States/x_dot -> x2/Hold this value ==
  In1 : Inport
  Action Port : ActionPort  ActionPortLabel=if(u1 ~= 0)
  Out1 : Outport  VectorParamsAs1DForOutWhenUnconnected=off
  wires:
  In1/1 -> Out1/1

== system CombinedExperiment/Grab PhaseSpace Data via UDP/Use Hardware to Obtain States/Using RED+BLACK, or RED+BLACK+ARM/Obtain BLACK States/x_dot -> x3/Hold this value ==
  In1 : Inport
  Action Port : ActionPort  ActionPortLabel=if(u1 ~= 0)
  Out1 : Outport  VectorParamsAs1DForOutWhenUnconnected=off
  wires:
  In1/1 -> Out1/1

== system CombinedExperiment/Grab PhaseSpace Data via UDP/Use Hardware to Obtain States/Using RED+BLACK, or RED+BLACK+ARM/Obtain BLACK States/x_dot -> x4/Hold this value ==
  In1 : Inport
  Action Port : ActionPort  ActionPortLabel=if(u1 ~= 0)
  Out1 : Outport  VectorParamsAs1DForOutWhenUnconnected=off
  wires:
  In1/1 -> Out1/1

== system CombinedExperiment/Grab PhaseSpace Data via UDP/Use Hardware to Obtain States/Using RED+BLACK, or RED+BLACK+ARM/Obtain BLACK States/x_dot -> x5/Hold this value ==
  In1 : Inport
  Action Port : ActionPort  ActionPortLabel=if(u1 ~= 0)
  Out1 : Outport  VectorParamsAs1DForOutWhenUnconnected=off
  wires:
  In1/1 -> Out1/1

== system CombinedExperiment/Grab PhaseSpace Data via UDP/Use Hardware to Obtain States/Using RED+BLACK, or RED+BLACK+ARM/Obtain BLACK States/x_dot -> x6/Hold this value ==
  In1 : Inport
  Action Port : ActionPort  ActionPortLabel=if(u1 ~= 0)
  Out1 : Outport  VectorParamsAs1DForOutWhenUnconnected=off
  wires:
  In1/1 -> Out1/1

== system CombinedExperiment/Grab PhaseSpace Data via UDP/Use Hardware to Obtain States/Using RED+BLACK, or RED+BLACK+ARM/Obtain BLACK States/x_dot -> x7/Hold this value ==
  In1 : Inport
  Action Port : ActionPort  ActionPortLabel=if(u1 ~= 0)
  Out1 : Outport  VectorParamsAs1DForOutWhenUnconnected=off
  wires:
  In1/1 -> Out1/1

== system CombinedExperiment/Grab PhaseSpace Data via UDP/Use Hardware to Obtain States/Using RED+BLACK, or RED+BLACK+ARM/Obtain BLACK States/x_dot -> x8/Hold this value ==
  In1 : Inport
  Action Port : ActionPort  ActionPortLabel=if(u1 ~= 0)
  Out1 : Outport  VectorParamsAs1DForOutWhenUnconnected=off
  wires:
  In1/1 -> Out1/1

== system CombinedExperiment/Grab PhaseSpace Data via UDP/Use Hardware to Obtain States/Using RED+BLACK, or RED+BLACK+ARM/Obtain BLACK States/x_dot -> x9/Hold this value ==
  In1 : Inport
  Action Port : ActionPort  ActionPortLabel=if(u1 ~= 0)
  Out1 : Outport  VectorParamsAs1DForOutWhenUnconnected=off
  wires:
  In1/1 -> Out1/1

== system CombinedExperiment/Grab PhaseSpace Data via UDP/Use Hardware to Obtain States/Using RED+BLACK, or RED+BLACK+ARM/Obtain RED States/Correct Time/Enabled Subsystem ==
  In1 : Inport
  Enable : EnablePort
  Out1 : Outport  VectorParamsAs1DForOutWhenUnconnected=off
  wires:
  In1/1 -> Out1/1

== system CombinedExperiment/Grab PhaseSpace Data via UDP/Use Hardware to Obtain States/Using RED+BLACK, or RED+BLACK+ARM/Obtain RED States/x_dot -> x1/Hold this value ==
  In1 : Inport
  Action Port : ActionPort  ActionPortLabel=if(u1 ~= 0)
  Out1 : Outport  VectorParamsAs1DForOutWhenUnconnected=off
  wires:
  In1/1 -> Out1/1

== system CombinedExperiment/Grab PhaseSpace Data via UDP/Use Hardware to Obtain States/Using RED+BLACK, or RED+BLACK+ARM/Obtain RED States/x_dot -> x10/Hold this value ==
  In1 : Inport
  Action Port : ActionPort  ActionPortLabel=if(u1 ~= 0)
  Out1 : Outport  VectorParamsAs1DForOutWhenUnconnected=off
  wires:
  In1/1 -> Out1/1

== system CombinedExperiment/Grab PhaseSpace Data via UDP/Use Hardware to Obtain States/Using RED+BLACK, or RED+BLACK+ARM/Obtain RED States/x_dot -> x11/Hold this value ==
  In1 : Inport
  Action Port : ActionPort  ActionPortLabel=if(u1 ~= 0)
  Out1 : Outport  VectorParamsAs1DForOutWhenUnconnected=off
  wires:
  In1/1 -> Out1/1

== system CombinedExperiment/Grab PhaseSpace Data via UDP/Use Hardware to Obtain States/Using RED+BLACK, or RED+BLACK+ARM/Obtain RED States/x_dot -> x12/Hold this value ==
  In1 : Inport
  Action Port : ActionPort  ActionPortLabel=if(u1 ~= 0)
  Out1 : Outport  VectorParamsAs1DForOutWhenUnconnected=off
  wires:
  In1/1 -> Out1/1

== system CombinedExperiment/Grab PhaseSpace Data via UDP/Use Hardware to Obtain States/Using RED+BLACK, or RED+BLACK+ARM/Obtain RED States/x_dot -> x2/Hold this value ==
  In1 : Inport
  Action Port : ActionPort  ActionPortLabel=if(u1 ~= 0)
  Out1 : Outport  VectorParamsAs1DForOutWhenUnconnected=off
  wires:
  In1/1 -> Out1/1

== system CombinedExperiment/Grab PhaseSpace Data via UDP/Use Hardware to Obtain States/Using RED+BLACK, or RED+BLACK+ARM/Obtain RED States/x_dot -> x3/Hold this value ==
  In1 : Inport
  Action Port : ActionPort  ActionPortLabel=if(u1 ~= 0)
  Out1 : Outport  VectorParamsAs1DForOutWhenUnconnected=off
  wires:
  In1/1 -> Out1/1

== system CombinedExperiment/Grab PhaseSpace Data via UDP/Use Hardware to Obtain States/Using RED+BLACK, or RED+BLACK+ARM/Obtain RED States/x_dot -> x4/Hold this value ==
  In1 : Inport
  Action Port : ActionPort  ActionPortLabel=if(u1 ~= 0)
  Out1 : Outport  VectorParamsAs1DForOutWhenUnconnected=off
  wires:
  In1/1 -> Out1/1

== system CombinedExperiment/Grab PhaseSpace Data via UDP/Use Hardware to Obtain States/Using RED+BLACK, or RED+BLACK+ARM/Obtain RED States/x_dot -> x5/Hold this value ==
  In1 : Inport
  Action Port : ActionPort  ActionPortLabel=if(u1 ~= 0)
  Out1 : Outport  VectorParamsAs1DForOutWhenUnconnected=off
  wires:
  In1/1 -> Out1/1

== system CombinedExperiment/Grab PhaseSpace Data via UDP/Use Hardware to Obtain States/Using RED+BLACK, or RED+BLACK+ARM/Obtain RED States/x_dot -> x6/Hold this value ==
  In1 : Inport
  Action Port : ActionPort  ActionPortLabel=if(u1 ~= 0)
  Out1 : Outport  VectorParamsAs1DForOutWhenUnconnected=off
  wires:
  In1/1 -> Out1/1

== system CombinedExperiment/Grab PhaseSpace Data via UDP/Use Hardware to Obtain States/Using RED+BLACK, or RED+BLACK+ARM/Obtain RED States/x_dot -> x7/Hold this value ==
  In1 : Inport
  Action Port : ActionPort  ActionPortLabel=if(u1 ~= 0)
  Out1 : Outport  VectorParamsAs1DForOutWhenUnconnected=off
  wires:
  In1/1 -> Out1/1

== system CombinedExperiment/Grab PhaseSpace Data via UDP/Use Hardware to Obtain States/Using RED+BLACK, or RED+BLACK+ARM/Obtain RED States/x_dot -> x8/Hold this value ==
  In1 : Inport
  Action Port : ActionPort  ActionPortLabel=if(u1 ~= 0)
  Out1 : Outport  VectorParamsAs1DForOutWhenUnconnected=off
  wires:
  In1/1 -> Out1/1

== system CombinedExperiment/Grab PhaseSpace Data via UDP/Use Hardware to Obtain States/Using RED+BLACK, or RED+BLACK+ARM/Obtain RED States/x_dot -> x9/Hold this value ==
  In1 : Inport
  Action Port : ActionPort  ActionPortLabel=if(u1 ~= 0)
  Out1 : Outport  VectorParamsAs1DForOutWhenUnconnected=off
  wires:
  In1/1 -> Out1/1

== system CombinedExperiment/Phase #3: Experiment/Change BLACK Behavior/Sub-Phase #1/Custom Discrete PD (Attitude)/x_dot -> x1/Hold this value ==
  In1 : Inport
  Action Port : ActionPort  ActionPortLabel=if(u1 ~= 0)
  Out1 : Outport  VectorParamsAs1DForOutWhenUnconnected=off
  wires:
  In1/1 -> Out1/1

== system CombinedExperiment/Phase #3: Experiment/Change BLACK Behavior/Sub-Phase #1/Custom Discrete PD (X-Position)/x_dot -> x1/Hold this value ==
  In1 : Inport
  Action Port : ActionPort  ActionPortLabel=if(u1 ~= 0)
  Out1 : Outport  VectorParamsAs1DForOutWhenUnconnected=off
  wires:
  In1/1 -> Out1/1

== system CombinedExperiment/Phase #3: Experiment/Change BLACK Behavior/Sub-Phase #1/Custom Discrete PD (Y-Position)/x_dot -> x1/Hold this value ==
  In1 : Inport
  Action Port : ActionPort  ActionPortLabel=if(u1 ~= 0)
  Out1 : Outport  VectorParamsAs1DForOutWhenUnconnected=off
  wires:
  In1/1 -> Out1/1

== system CombinedExperiment/Phase #3: Experiment/Change BLACK Behavior/Sub-Phase #4/Custom Discrete PD (Attitude)/x_dot -> x1/Hold this value ==
  In1 : Inport
  Action Port : ActionPort  ActionPortLabel=if(u1 ~= 0)
  Out1 : Outport  VectorParamsAs1DForOutWhenUnconnected=off
  wires:
  In1/1 -> Out1/1

== system CombinedExperiment/Phase #3: Experiment/Change BLACK Behavior/Sub-Phase #4/Custom Discrete PD (X-Position)/x_dot -> x1/Hold this value ==
  In1 : Inport
  Action Port : ActionPort  ActionPortLabel=if(u1 ~= 0)
  Out1 : Outport  VectorParamsAs1DForOutWhenUnconnected=off
  wires:
  In1/1 -> Out1/1

== system CombinedExperiment/Phase #3: Experiment/Change BLACK Behavior/Sub-Phase #4/Custom Discrete PD (Y-Position)/x_dot -> x1/Hold this value ==
  In1 : Inport
  Action Port : ActionPort  ActionPortLabel=if(u1 ~= 0)
  Out1 : Outport  VectorParamsAs1DForOutWhenUnconnected=off
  wires:
  In1/1 -> Out1/1

== system CombinedExperiment/Phase #3: Experiment/Change BLUE Behavior/Sub-Phase #1/Custom Discrete PD (Attitude)/x_dot -> x1/Hold this value ==
  In1 : Inport
  Action Port : ActionPort  ActionPortLabel=if(u1 ~= 0)
  Out1 : Outport  VectorParamsAs1DForOutWhenUnconnected=off
  wires:
  In1/1 -> Out1/1

== system CombinedExperiment/Phase #3: Experiment/Change BLUE Behavior/Sub-Phase #1/Custom Discrete PD (X-Position)/x_dot -> x1/Hold this value ==
  In1 : Inport
  Action Port : ActionPort  ActionPortLabel=if(u1 ~= 0)
  Out1 : Outport  VectorParamsAs1DForOutWhenUnconnected=off
  wires:
  In1/1 -> Out1/1

== system CombinedExperiment/Phase #3: Experiment/Change BLUE Behavior/Sub-Phase #1/Custom Discrete PD (Y-Position)/x_dot -> x1/Hold this value ==
  In1 : Inport
  Action Port : ActionPort  ActionPortLabel=if(u1 ~= 0)
  Out1 : Outport  VectorParamsAs1DForOutWhenUnconnected=off
  wires:
  In1/1 -> Out1/1

== system CombinedExperiment/Phase #3: Experiment/Change BLUE Behavior/Sub-Phase #4/Custom Discrete PD (Attitude)/x_dot -> x1/Hold this value ==
  In1 : Inport
  Action Port : ActionPort  ActionPortLabel=if(u1 ~= 0)
  Out1 : Outport  VectorParamsAs1DForOutWhenUnconnected=off
  wires:
  In1/1 -> Out1/1

== system CombinedExperiment/Phase #3: Experiment/Change BLUE Behavior/Sub-Phase #4/Custom Discrete PD (X-Position)/x_dot -> x1/Hold this value ==
  In1 : Inport
  Action Port : ActionPort  ActionPortLabel=if(u1 ~= 0)
  Out1 : Outport  VectorParamsAs1DForOutWhenUnconnected=off
  wires:
  In1/1 -> Out1/1

== system CombinedExperiment/Phase #3: Experiment/Change BLUE Behavior/Sub-Phase #4/Custom Discrete PD (Y-Position)/x_dot -> x1/Hold this value ==
  In1 : Inport
  Action Port : ActionPort  ActionPortLabel=if(u1 ~= 0)
  Out1 : Outport  VectorParamsAs1DForOutWhenUnconnected=off
  wires:
  In1/1 -> Out1/1

== system CombinedExperiment/Phase #3: Experiment/Change RED Behavior/Sub-Phase #4/Custom Discrete PD (Attitude)2/x_dot -> x1/Hold this value ==
  In1 : Inport
  Action Port : ActionPort  ActionPortLabel=if(u1 ~= 0)
  Out1 : Outport  VectorParamsAs1DForOutWhenUnconnected=off
  wires:
  In1/1 -> Out1/1

== matlab function CombinedExperiment/From Force//Torque to PWM Signal/Change BLACK Behavior/Calculate Thruster ON//OFF/MATLAB Function ==
  data: H output; thruster_dist2CG_BLACK parameter; F_thrusters_BLACK parameter
function H = MakeH(thruster_dist2CG_BLACK,F_thrusters_BLACK)

Vec1 = [ -1
         -1
          0 
          0
          1
          1
          0
          0 ];
      
Vec2 = [  0
          0
          1
          1
          0
          0
         -1
         -1 ];
     
Vec3 = thruster_dist2CG_BLACK./1000;

Mat1 = [Vec1, Vec2, Vec3]';

Mat2 = diag((F_thrusters_BLACK./2));

H    = Mat1*Mat2;

end

== matlab function CombinedExperiment/Phase #3: Experiment/Change BLACK Behavior/Sub-Phase #4/BLACK_RzD/Wrap1/MATLAB Function ==
  data: u input; wrappedAngle output
function wrappedAngle = wrapAngle(u)

wrappedAngle = atan2(sin(u),cos(u));

end

== matlab function CombinedExperiment/Phase #3: Experiment/Change BLACK Behavior/Sub-Phase #4/Hough Control/MATLAB Function2 ==
  data: Oy output; z input; Ox output
function [Oy, Ox]   = C3( z )
%C3 gives the rotation matrix about the z-axis for an angle 'z'
%   z - the angle about the z-axis which you rotate
%   A - the rotation matrix

Ox = [cos(z) sin(z); -sin(z) cos(z)]*[1;0];
Oy = [cos(z) sin(z); -sin(z) cos(z)]*[0;1];
end

== matlab function CombinedExperiment/From Force//Torque to PWM Signal/Change BLACK Behavior/Calculate Thruster ON//OFF/MATLAB Function1 ==
  data: H output; thruster_dist2CG_BLACK parameter; F_thrusters_BLACK parameter
function H = MakeH(thruster_dist2CG_BLACK,F_thrusters_BLACK)

Vec1 = [ -1
         -1
          0 
          0
          1
          1
          0
          0 ];
      
Vec2 = [  0
          0
          1
          1
          0
          0
         -1
         -1 ];
     
Vec3 = thruster_dist2CG_BLACK./1000;

Mat1 = [Vec1, Vec2, Vec3]';

Mat2 = diag((F_thrusters_BLACK));

H    = Mat1*Mat2;

end

== matlab function CombinedExperiment/From Force//Torque to PWM Signal/Change BLACK Behavior/Calculate Thruster ON//OFF/MATLAB Function2 ==
  data: ThrustPer_Final output; ThrustPer input
function ThrustPer_Final  = ThrusterSat(ThrustPer)

ValveTime       = 0.007;
TControl        = 0.1;
ThrustPer_Final = zeros(8,1);

if max(ThrustPer) > 1
    ThrustPer_Sat = ThrustPer/max(ThrustPer);
else
    ThrustPer_Sat = ThrustPer;
end

for i = 1:8
    if ThrustPer_Sat(i) > ValveTime/TControl 
        ThrustPer_Final(i) = ThrustPer_Sat(i);
    else
        ThrustPer_Final(i) = 0;
    end
end
   

end
